simulink model "VehicleDynamics"  (R2025b)
settings: Solver=FixedStepAuto  StartTime=0.0  StopTime=25  FixedStep=0.001  RelTol=1e-3
PreLoadFcn:
  | vehicle_parameters
values from neighbouring files (symbols this model uses):
  beta0 = 0    [vehicle_parameters.m]
  drag = 0    [vehicle_parameters.m]
  ff = 0    [vehicle_parameters.m]
  Fmax = 1274.11    [vehicle_parameters.m]
  N = 15    [MPC_script.m]
  psi0 = 0    [vehicle_parameters.m]
  psi_dot0 = 0    [vehicle_parameters.m]
  RoadCond = 0    [vehicle_parameters.m]
  theta = deg2rad(theta)    [LinearModel.m]    (also in NonLinearModel.m; vehicle_parameters.m = 0)
  vx0 = 0.1    [vehicle_parameters.m]
  vx_constant = 10    [vehicle_parameters.m]
  w = omega_ref    [Fx_w_map.m]
  x0 = 0    [vehicle_parameters.m]
  y0 = 0    [vehicle_parameters.m]
undefined symbols (not defined in the file or in its folder): feedforward, Fx_w_map, K, LinearModel, model, MPC, NonLinearModel, Orientation, Saturation
libraries: slpidlib x1
settings Model: Creator=School  LastModifiedBy=School

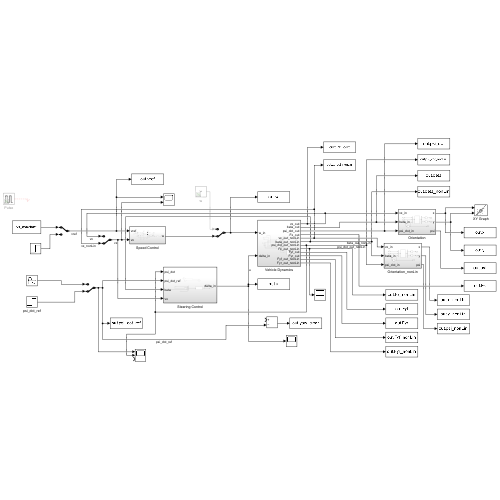
[thumbnail: Simulink's stored preview of the top-level diagram]
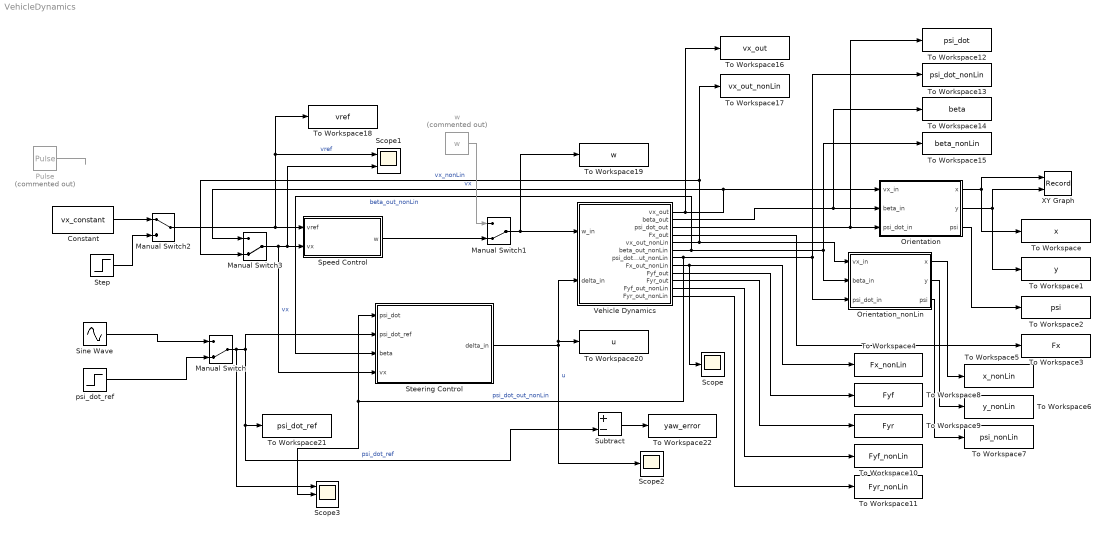
== system VehicleDynamics ==
  Constant : Constant  Value=vx_constant
  Manual Switch : ManualSwitch  CurrentSetting=0
  Manual Switch1 : ManualSwitch  CurrentSetting=0
  Manual Switch2 : ManualSwitch
  Manual Switch3 : ManualSwitch  CurrentSetting=0
  Orientation : Subsystem
  Orientation_nonLin : Subsystem
  Pulse : DiscretePulseGenerator  Commented=on  PulseType=Time based  Amplitude=25  Period=20  PulseWidth=50
  Scope : Scope
      settings: ActiveDisplayYMinimum=-980.76800111578189  ActiveDisplayYMaximum=7754.1424627217448  DataLoggingVariableName=ScopeData5
  Scope1 : Scope  NumInputPorts=2
      settings: ActiveDisplayYMinimum=-1.3886045120699795  ActiveDisplayYMaximum=13.49744060862982  DataLoggingVariableName=ScopeData6
  Scope2 : Scope
      settings: ActiveDisplayYMinimum=-0.012691379481544529  ActiveDisplayYMaximum=0.081489371948126221  DataLoggingVariableName=ScopeData12
  Scope3 : Scope  NumInputPorts=3
      settings: ActiveDisplayYMinimum=-0.011480391205702918  ActiveDisplayYMaximum=0.098238335244763081  DataLoggingVariableName=ScopeData13
  Sine Wave : Sin  Amplitude=deg2rad(5)  Frequency=0.2  SampleTime=0
  Speed Control : Subsystem
  Steering Control : Subsystem
  Step : Step  Time=0  After=10  SampleTime=0
  Subtract : Sum  Inputs=+-
  To Workspace : ToWorkspace  VariableName=x  SaveFormat=Timeseries  SampleTime=-1
  To Workspace1 : ToWorkspace  VariableName=y  SaveFormat=Timeseries  SampleTime=-1
  To Workspace10 : ToWorkspace  VariableName=Fyf_nonLin  SaveFormat=Timeseries  SampleTime=-1
  To Workspace11 : ToWorkspace  VariableName=Fyr_nonLin  SaveFormat=Timeseries  SampleTime=-1
  To Workspace12 : ToWorkspace  VariableName=psi_dot  SaveFormat=Timeseries  SampleTime=-1
  To Workspace13 : ToWorkspace  VariableName=psi_dot_nonLin  SaveFormat=Timeseries  SampleTime=-1
  To Workspace14 : ToWorkspace  VariableName=beta  SaveFormat=Timeseries  SampleTime=-1
  To Workspace15 : ToWorkspace  VariableName=beta_nonLin  SaveFormat=Timeseries  SampleTime=-1
  To Workspace16 : ToWorkspace  VariableName=vx_out  SaveFormat=Timeseries  SampleTime=-1
  To Workspace17 : ToWorkspace  VariableName=vx_out_nonLin  SaveFormat=Timeseries  SampleTime=-1
  To Workspace18 : ToWorkspace  VariableName=vref  SaveFormat=Timeseries  SampleTime=-1
  To Workspace19 : ToWorkspace  VariableName=w  SaveFormat=Timeseries  SampleTime=-1
  To Workspace2 : ToWorkspace  VariableName=psi  SaveFormat=Timeseries  SampleTime=-1
  To Workspace20 : ToWorkspace  VariableName=u  SaveFormat=Timeseries  SampleTime=-1
  To Workspace21 : ToWorkspace  VariableName=psi_dot_ref  SaveFormat=Timeseries  SampleTime=-1
  To Workspace22 : ToWorkspace  VariableName=yaw_error  SaveFormat=Timeseries  SampleTime=-1
  To Workspace3 : ToWorkspace  VariableName=Fx  SaveFormat=Timeseries  SampleTime=-1
  To Workspace4 : ToWorkspace  VariableName=Fx_nonLin  SaveFormat=Timeseries  SampleTime=-1
  To Workspace5 : ToWorkspace  VariableName=x_nonLin  SaveFormat=Timeseries  SampleTime=-1
  To Workspace6 : ToWorkspace  VariableName=y_nonLin  SaveFormat=Timeseries  SampleTime=-1
  To Workspace7 : ToWorkspace  VariableName=psi_nonLin  SaveFormat=Timeseries  SampleTime=-1
  To Workspace8 : ToWorkspace  VariableName=Fyf  SaveFormat=Timeseries  SampleTime=-1
  To Workspace9 : ToWorkspace  VariableName=Fyr  SaveFormat=Timeseries  SampleTime=-1
  Vehicle Dynamics : Subsystem
  XY Graph : Record  NumPorts=2.0  FileSettingsInternal="{\"entries\":[{\"content\":{\"excelSettings\":{\"content\":{},\"type\":\"Streamout.ExcelSettings\"},\"parquetSettings\":{\"content\":{},\"type\":\"Streamout.ParquetSettings\"}},\"type\":\"Streamout.FileSettingStorage\",\"uuid\":\"\"}],\"packageUris\":[\"http:\\/\\/schema.mathworks.com\\/mf0\\/streamout_blocks\\/R2020a\"],\"version\":\"1.0\"}"  FrameSettings=[0, 0]  Layout=[1 1]  SignalsInternal="{\"entries\":[{\"content\":{\"signals\":[{\"content\":{\"blockPath\":[],\"dimensions\":[1,1],\"domain\":\"\",\"lineColor\":\"#ff13a6\",\"lineWidth\":2,\"plots\":[ 1 ],\"port\":1,\"sid\":[\"\"],\"signalID\":1,\"signalName\":\"Orientation:1\"},\"type\":\"RecordBlkView.Signal\",\"uuid\":\"\"},{\"content\":{\"blockPath\":[],\"dimensions\":[1,1],\"domain\":\"\",\"lineColor\":\"#fe330a\",\"lineWidth\":2,\"plots\":[ 1 ],\"port\":2,\"sid\":[\"\"],\"signalID\":2,\"signalName\":\"Orientation:2\"},\"type\":\"RecordBlkView.Signal\",\"uuid\":\"\"}]},\"type\":\"RecordBlkView.InputSignals\",\"uuid\":\"\"}],\"packageUris\":[\"http:\\/\\/schema.mathworks.com\\/mf0\\/streamout_blocks\\/R2020a\"],\"version\":\"1.0\"}"  VisualizationBindings="{\"xyplotplugin\":{\"info\":[{\"series\":[{\"bindingParametersList\":[{\"parameter\":\"X-Axis\",\"signalID\":1,\"signalName\":\"Orientation:1\"},{\"parameter\":\"Y-Axis\",\"signalID\":2,\"signalName\":\"Orientation:2\"}],\"seriesID\":0}],\"subplotID\":1}]}}"  CompatibilityTag=XY
  psi_dot_ref : Step  Time=15  After=deg2rad(5)  SampleTime=0
  w : Constant  Commented=on  Value=w
  wires:
  Vehicle Dynamics/1(vx_out) -> To Workspace16/1, Orientation/1(vx_in), Manual Switch3/1  "vx"
  Vehicle Dynamics/2(beta_out) -> Orientation/2(beta_in), To Workspace14/1
  Vehicle Dynamics/3(psi_dot_out) -> To Workspace12/1, Orientation/3(psi_dot_in)
  Orientation/1(x) -> XY Graph/1, To Workspace/1
  Orientation/2(y) -> XY Graph/2, To Workspace1/1
  Orientation/3(psi) -> To Workspace2/1
  Vehicle Dynamics/4(Fx_out) -> To Workspace3/1
  Vehicle Dynamics/5(vx_out_nonLin) -> Manual Switch3/2, To Workspace17/1, Orientation_nonLin/1(vx_in)  "vx_nonLin"
  Vehicle Dynamics/6(beta_out_nonLin) -> Steering Control/3(beta), To Workspace15/1, Orientation_nonLin/2(beta_in)  "beta_out_nonLin"
  Vehicle Dynamics/7(psi_dot_out_nonLin) -> Scope3/2, Steering Control/1(psi_dot), To Workspace13/1, Orientation_nonLin/3(psi_dot_in)  "psi_dot_out_nonLin"
  Vehicle Dynamics/8(Fx_out_nonLin) -> Scope/1, To Workspace4/1
  Orientation_nonLin/1(x) -> To Workspace5/1
  Orientation_nonLin/2(y) -> To Workspace6/1
  Orientation_nonLin/3(psi) -> To Workspace7/1
  Vehicle Dynamics/9(Fyf_out) -> To Workspace8/1
  Vehicle Dynamics/10(Fyr_out) -> To Workspace9/1
  Vehicle Dynamics/11(Fyf_out_nonLin) -> To Workspace10/1
  Vehicle Dynamics/12(Fyr_out_nonLin) -> To Workspace11/1
  psi_dot_ref/1 -> Manual Switch/2
  w/1 -> Manual Switch1/1
  Manual Switch1/1 -> To Workspace19/1, Vehicle Dynamics/1(w_in)
  Speed Control/1(w) -> Manual Switch1/2
  Pulse/1 -> ?
  Step/1 -> Manual Switch2/2
  Manual Switch3/1 -> Steering Control/4(vx), Scope1/2, Speed Control/2(vx)  "vx"
  Manual Switch2/1 -> Speed Control/1(vref), To Workspace18/1, Scope1/1  "vref"
  Steering Control/1(delta_in) -> Vehicle Dynamics/2(delta_in), To Workspace20/1, Scope2/1  "u"
  Manual Switch/1 -> Scope3/1, Subtract/2, To Workspace21/1, Steering Control/2(psi_dot_ref)  "psi_dot_ref"
  Constant/1 -> Manual Switch2/1
  Subtract/1 -> To Workspace22/1
  Sine Wave/1 -> Manual Switch/1

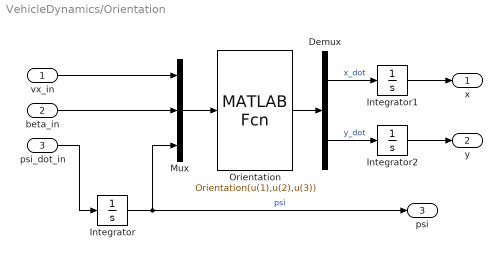
== system VehicleDynamics/Orientation ==
  vx_in : Inport
  beta_in : Inport  Port=2
  psi_dot_in : Inport  Port=3
  Demux : Demux  Outputs=2
  Integrator : Integrator  InitialCondition=psi0
  Integrator1 : Integrator  InitialCondition=x0
  Integrator2 : Integrator  InitialCondition=y0
  Mux : Mux  Inputs=3
  Orientation : MATLABFcn  MATLABFcn=Orientation(u(1),u(2),u(3))  OutputDimensions=[2,1]  Output1D=off
  x : Outport
  y : Outport  Port=2
  psi : Outport  Port=3
  wires:
  Mux/1 -> Orientation/1
  vx_in/1 -> Mux/1
  beta_in/1 -> Mux/2
  Demux/1 -> Integrator1/1  "x_dot"
  Demux/2 -> Integrator2/1  "y_dot"
  Orientation/1 -> Demux/1
  psi_dot_in/1 -> Integrator/1
  Integrator/1 -> Mux/3, psi/1  "psi"
  Integrator2/1 -> y/1
  Integrator1/1 -> x/1

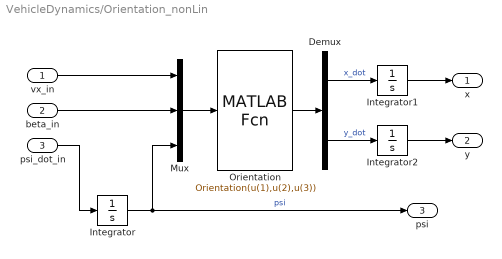
== system VehicleDynamics/Orientation_nonLin ==
  vx_in : Inport
  beta_in : Inport  Port=2
  psi_dot_in : Inport  Port=3
  Demux : Demux  Outputs=2
  Integrator : Integrator  InitialCondition=psi0
  Integrator1 : Integrator  InitialCondition=x0
  Integrator2 : Integrator  InitialCondition=y0
  Mux : Mux  Inputs=3
  Orientation : MATLABFcn  MATLABFcn=Orientation(u(1),u(2),u(3))  OutputDimensions=[2,1]  Output1D=off
  x : Outport
  y : Outport  Port=2
  psi : Outport  Port=3
  wires:
  Mux/1 -> Orientation/1
  vx_in/1 -> Mux/1
  beta_in/1 -> Mux/2
  Demux/1 -> Integrator1/1  "x_dot"
  Demux/2 -> Integrator2/1  "y_dot"
  Orientation/1 -> Demux/1
  psi_dot_in/1 -> Integrator/1
  Integrator/1 -> Mux/3, psi/1  "psi"
  Integrator2/1 -> y/1
  Integrator1/1 -> x/1

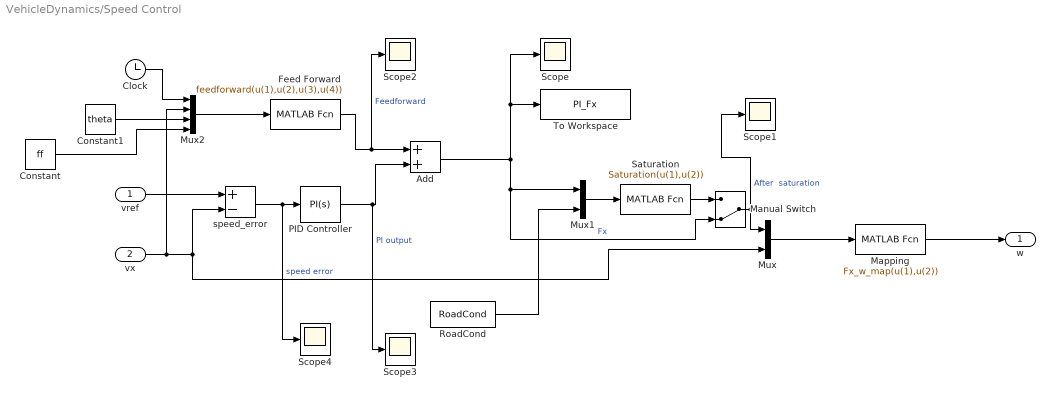
== system VehicleDynamics/Speed Control ==
  vref : Inport
  vx : Inport  Port=2
  Add : Sum
  Clock : Clock
  Constant : Constant  Value=ff
  Constant1 : Constant  Value=theta
  Feed Forward : MATLABFcn  MATLABFcn=feedforward(u(1),u(2),u(3),u(4))  OutputDimensions=1  Output1D=off
  Manual Switch : ManualSwitch  CurrentSetting=0
  Mapping : MATLABFcn  MATLABFcn=Fx_w_map(u(1),u(2))  OutputDimensions=[1,1]  Output1D=off
  Mux : Mux  Inputs=2
  Mux1 : Mux  Inputs=2
  Mux2 : Mux
  PID Controller : slpidlib/PID Controller  Controller=PI  Form=Parallel  TimeDomain=Continuous-time  UseExternalTs=off  SampleTime=-1  IntegratorMethod=Forward Euler  FilterMethod=Forward Euler  ControllerParametersSource=internal  P=4*206  I=206  UseKiTs=off  D=0  UseExternalDerivativeSource=off  N=100  UseFilter=on  TunerSelectOption=Transfer Function Based (PID Tuner App)  InitialConditionSource=internal  InitialConditionForIntegrator=0  InitialConditionForFilter=0  DifferentiatorICPrevScaledInput=0  ExternalReset=none  TrackingMode=off  Kt=1  LimitOutput=on  SatLimitsSource=internal  UpperSaturationLimit=Fmax  LowerSaturationLimit=-Fmax  LinearizeAsGain=off  AntiWindupMode=back-calculation  Kb=206/(4*206)  LimitIntegrator=off  UpperIntegratorSaturationLimit=inf  LowerIntegratorSaturationLimit=-inf  POutMin=[]  POutMax=[]  IOutMin=[]  IOutMax=[]  DOutMin=[]  DOutMax=[]  NOutMin=[]  NOutMax=[]  SumOutMin=[]  SumOutMax=[]  SaturationOutMin=[]  SaturationOutMax=[]  PParamMin=[]  PParamMax=[]  IParamMin=[]  IParamMax=[]  DParamMin=[]  DParamMax=[]  NParamMin=[]  NParamMax=[]  KbParamMin=[]  KbParamMax=[]  KtParamMin=[]  KtParamMax=[]  KbOutMin=[]  KbOutMax=[]  KtOutMin=[]  KtOutMax=[]  IntegratorOutMin=[]  IntegratorOutMax=[]  FilterOutMin=[]  FilterOutMax=[]  SumI1OutMin=[]  SumI1OutMax=[]  SumI2OutMin=[]  SumI2OutMax=[]  SumI3OutMin=[]  SumI3OutMax=[]  SumI4OutMin=[]  SumI4OutMax=[]  SumDOutMin=[]  SumDOutMax=[]  DifferentiatorOutMin=[]  DifferentiatorOutMax=[]  FilterDiffOutCoefMin=[]  FilterDiffOutCoefMax=[]  ReciprocalOutMin=[]  ReciprocalOutMax=[]  SumDenOutMin=[]  SumDenOutMax=[]  SumNumOutMin=[]  SumNumOutMax=[]  DivideOutMin=[]  DivideOutMax=[]  UdiffTsProdOutMin=[]  UdiffTsProdOutMax=[]  NTsProdOutMin=[]  NTsProdOutMax=[]  UintegralTsProdOutMin=[]  UintegralTsProdOutMax=[]  UngainTsProdOutMin=[]  UngainTsProdOutMax=[]  ClampingZeroOutDataTypeStr=Inherit: Inherit via back propagation  ClampingZeroOutMin=[]  ClampingZeroOutMax=[]  FilterDenConstantOutDataTypeStr=Inherit: Inherit via back propagation  FilterDenConstantOutMin=[]  FilterDenConstantOutMax=[]  PCopyOutDataTypeStr=Inherit: Inherit via back propagation  PCopyOutMin=[]  PCopyOutMax=[]  NCopyOutDataTypeStr=Inherit: Inherit via back propagation  NCopyOutMin=[]  NCopyOutMax=[]  IntegratorContinuousStateAttributes=''  IntegratorStateMustResolveToSignalObject=off  IntegratorRTWStateStorageClass=Auto  FilterContinuousStateAttributes=''  FilterStateMustResolveToSignalObject=off  FilterRTWStateStorageClass=Auto  ParallelPVariant=InternalParameters  IdealPVariant=Disabled  IVariant=InternalParameters  DVariant=Disabled  IntegratorVariant=Continuous  SatVariant=Enabled  AWVariant=BackCalculation  PCopyVariant=Disabled  TRVariant=Disabled  FdbkBlocksVariant=Forward  IdealPFdbkVariant=Disabled  SatFdbkVariant=Disabled  DerivativeFilterVariant=Disabled  NVariant=Disabled  NCopyVariant=Disabled_SignalSpec  FilterICVariant=Disabled  IntegratorICVariant=InternalICs  ExternalResetVariant=Disabled  TRSumVariant=Passthrough  SumFdbkVariant=Disabled  SumVariant=Sum_PI  TsampFilterVariant=InternalTs  TsampNgainVariant=Passthrough  TsampIntegralVariant=Disabled_SignalSpec  ExternalSaturationOutDataTypeStr=Inherit: Same as second input  DerivativeSourceVariant=Disabled  PreIntVariant=InternalPreInt
  RoadCond : Constant  Value=RoadCond
  Saturation : MATLABFcn  MATLABFcn=Saturation(u(1),u(2))  OutputDimensions=1  Output1D=off
  Scope{,1..4} (5 alike) : Scope
      Scope settings: ActiveDisplayYMinimum=-1555.3315998720143  ActiveDisplayYMaximum=12511.361836654254  DataLoggingVariableName=ScopeData7
      Scope1 settings: ActiveDisplayYMinimum=-1027.3262882468107  ActiveDisplayYMaximum=7759.3140320274233  DataLoggingVariableName=ScopeData8
      Scope2 settings: ActiveDisplayYMinimum=1496.5482656031122  ActiveDisplayYMaximum=2205.6055136294681  DataLoggingVariableName=ScopeData9
      Scope3 settings: ActiveDisplayYMinimum=-2981.7756192687925  ActiveDisplayYMaximum=7976.4750688076438  DataLoggingVariableName=ScopeData10
      Scope4 settings: ActiveDisplayYMinimum=-10.514371710749185  ActiveDisplayYMaximum=34.390485745638792  DataLoggingVariableName=ScopeData11
  To Workspace : ToWorkspace  VariableName=PI_Fx  SaveFormat=Timeseries  SampleTime=-1
  speed_error : Sum  Inputs=+-
  w : Outport
  wires:
  vref/1 -> speed_error/1
  vx/1 -> Mux2/2, Mux/2, speed_error/2
  speed_error/1 -> PID Controller/1, Scope4/1  "speed error"
  Mux/1 -> Mapping/1
  Mapping/1 -> w/1
  Mux1/1 -> Saturation/1
  RoadCond/1 -> Mux1/2
  Saturation/1 -> Manual Switch/1
  Manual Switch/1 -> Mux/1, Scope1/1  "After  saturation"
  PID Controller/1 -> Scope3/1, Add/2  "PI output"
  Add/1 -> Scope/1, To Workspace/1, Manual Switch/2, Mux1/1  "Fx"
  Feed Forward/1 -> Scope2/1, Add/1  "Feedforward"
  Constant/1 -> Mux2/4
  Mux2/1 -> Feed Forward/1
  Clock/1 -> Mux2/1
  Constant1/1 -> Mux2/3

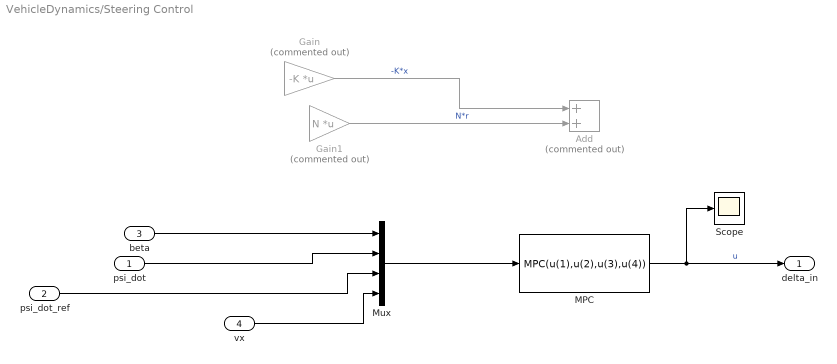
== system VehicleDynamics/Steering Control ==
  psi_dot : Inport
  psi_dot_ref : Inport  Port=2
  beta : Inport  Port=3
  vx : Inport  Port=4
  Add : Sum  Commented=on
  Gain : Gain  Commented=on  Gain=-K  Multiplication=Matrix(K*u)
  Gain1 : Gain  Commented=on  Gain=N  Multiplication=Matrix(K*u)
  MPC : MATLABFcn  MATLABFcn=MPC(u(1),u(2),u(3),u(4))  OutputDimensions=1  Output1D=off
  Mux : Mux
  Scope : Scope
      settings: ActiveDisplayYMinimum=-1  ActiveDisplayYMaximum=1  DataLoggingVariableName=ScopeData14
  delta_in : Outport
  wires:
  psi_dot/1 -> Mux/2
  beta/1 -> Mux/1
  Gain/1 -> Add/1  "-K*x"
  Gain1/1 -> Add/2  "N*r"
  MPC/1 -> Scope/1, delta_in/1  "u"
  psi_dot_ref/1 -> Mux/3
  vx/1 -> Mux/4
  Mux/1 -> MPC/1

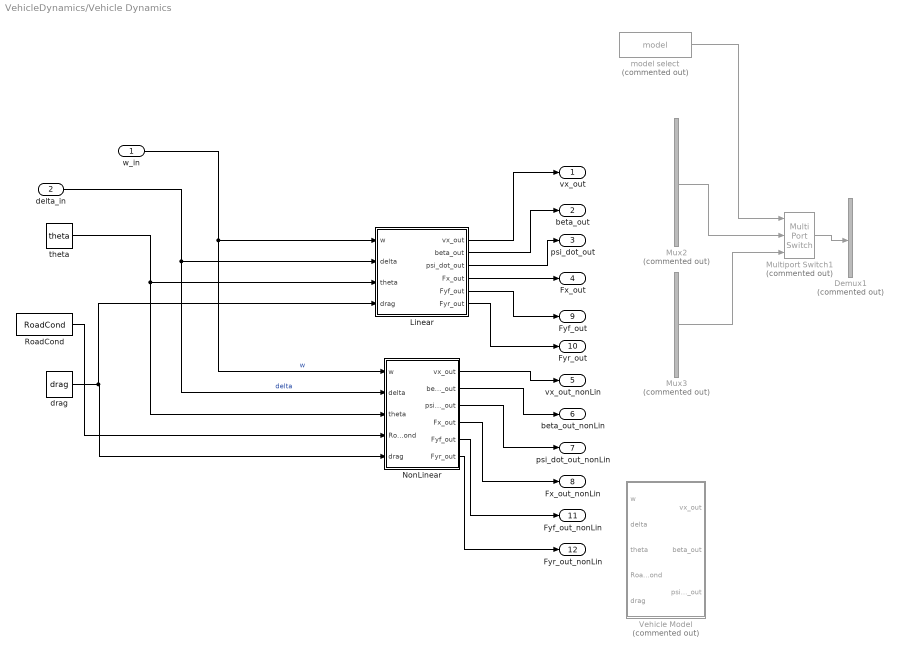
== system VehicleDynamics/Vehicle Dynamics ==
  w_in : Inport
  delta_in : Inport  Port=2
  Demux1 : Demux  Commented=on
  Linear : Subsystem
  Multiport Switch1 : MultiPortSwitch  Commented=on  Inputs=2  SaturateOnIntegerOverflow=off  InputSameDT=off
  Mux2 : Mux  Commented=on
  Mux3 : Mux  Commented=on
  NonLinear : Subsystem
  RoadCond : Constant  Value=RoadCond
  Vehicle Model : Subsystem  Commented=on  Variant=on
  drag : Constant  Value=drag
  model select : Constant  Commented=on  Value=model
  theta : Constant  Value=theta
  vx_out : Outport
  beta_out : Outport  Port=2
  psi_dot_out : Outport  Port=3
  Fx_out : Outport  Port=4
  vx_out_nonLin : Outport  Port=5
  beta_out_nonLin : Outport  Port=6
  psi_dot_out_nonLin : Outport  Port=7
  Fx_out_nonLin : Outport  Port=8
  Fyf_out : Outport  Port=9
  Fyr_out : Outport  Port=10
  Fyf_out_nonLin : Outport  Port=11
  Fyr_out_nonLin : Outport  Port=12
  wires:
  w_in/1 -> NonLinear/1(w), Linear/1(w)  "w"
  delta_in/1 -> NonLinear/2(delta), Linear/2(delta)  "delta"
  theta/1 -> NonLinear/3(theta), Linear/3(theta)
  RoadCond/1 -> NonLinear/4(RoadCond)
  drag/1 -> Linear/4(drag), NonLinear/5(drag)
  Multiport Switch1/1 -> Demux1/1
  model select/1 -> Multiport Switch1/1
  Mux2/1 -> Multiport Switch1/2
  Mux3/1 -> Multiport Switch1/3
  Linear/1(vx_out) -> vx_out/1
  Linear/2(beta_out) -> beta_out/1
  Linear/3(psi_dot_out) -> psi_dot_out/1
  Linear/4(Fx_out) -> Fx_out/1
  NonLinear/1(vx_out) -> vx_out_nonLin/1
  NonLinear/2(beta_out) -> beta_out_nonLin/1
  NonLinear/3(psi_dot_out) -> psi_dot_out_nonLin/1
  NonLinear/4(Fx_out) -> Fx_out_nonLin/1
  Linear/5(Fyf_out) -> Fyf_out/1
  Linear/6(Fyr_out) -> Fyr_out/1
  NonLinear/5(Fyf_out) -> Fyf_out_nonLin/1
  NonLinear/6(Fyr_out) -> Fyr_out_nonLin/1

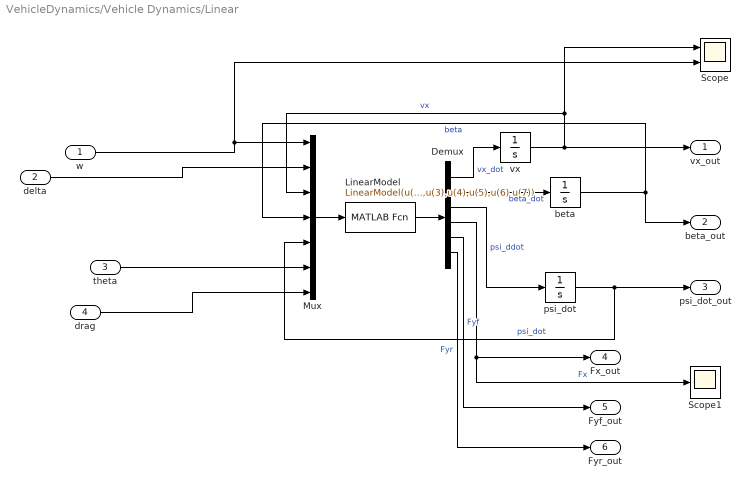
== system VehicleDynamics/Vehicle Dynamics/Linear ==
  w : Inport
  delta : Inport  Port=2
  theta : Inport  Port=3
  drag : Inport  Port=4
  Demux : Demux  Outputs=6
  LinearModel : MATLABFcn  MATLABFcn=LinearModel(u(1),u(2),u(3),u(4),u(5),u(6),u(7))  OutputDimensions=[6,1]  Output1D=off
  Mux : Mux  Inputs=7
  Scope : Scope  NumInputPorts=2
      settings: ActiveDisplayYMinimum=-3.6374999999999993  ActiveDisplayYMaximum=33.7375  DataLoggingVariableName=ScopeData2
  Scope1 : Scope
      settings: ActiveDisplayYMinimum=-735634.97602375317  ActiveDisplayYMaximum=6.61829277511375E+6  DataLoggingVariableName=ScopeData3
  beta : Integrator  InitialCondition=beta0
  psi_dot : Integrator  InitialCondition=psi_dot0
  vx : Integrator  InitialCondition=vx0
  vx_out : Outport
  beta_out : Outport  Port=2
  psi_dot_out : Outport  Port=3
  Fx_out : Outport  Port=4
  Fyf_out : Outport  Port=5
  Fyr_out : Outport  Port=6
  wires:
  delta/1 -> Mux/2
  w/1 -> Scope/2, Mux/1
  psi_dot/1 -> psi_dot_out/1, Mux/5  "psi_dot"
  LinearModel/1 -> Demux/1
  vx/1 -> vx_out/1, Scope/1, Mux/3  "vx"
  Demux/1 -> vx/1  "vx_dot"
  Demux/2 -> beta/1  "beta_dot"
  theta/1 -> Mux/6
  drag/1 -> Mux/7
  Mux/1 -> LinearModel/1
  Demux/3 -> psi_dot/1  "psi_ddot"
  beta/1 -> beta_out/1, Mux/4  "beta"
  Demux/4 -> Scope1/1, Fx_out/1  "Fx"
  Demux/5 -> Fyf_out/1  "Fyf"
  Demux/6 -> Fyr_out/1  "Fyr"

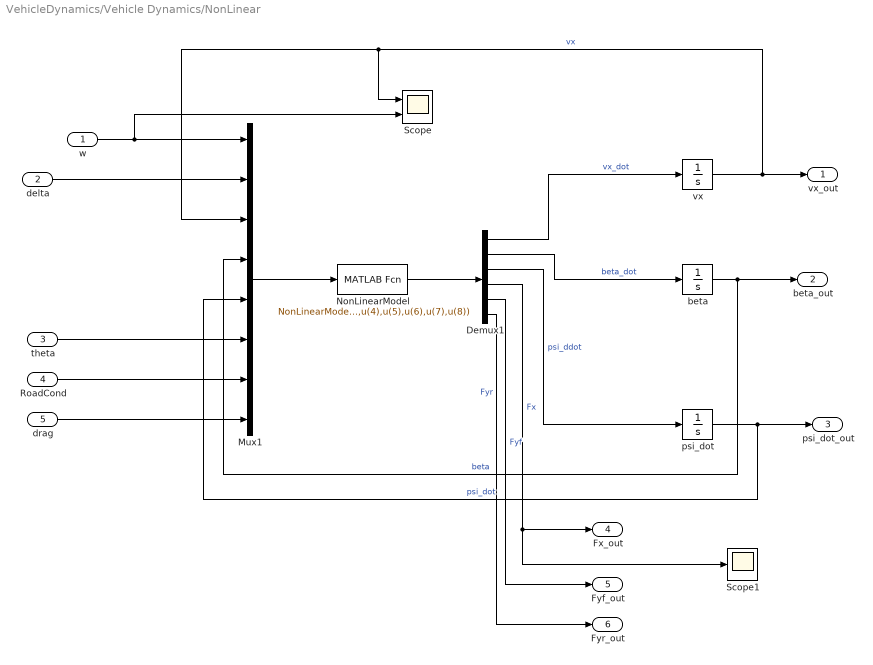
== system VehicleDynamics/Vehicle Dynamics/NonLinear ==
  w : Inport
  delta : Inport  Port=2
  theta : Inport  Port=3
  RoadCond : Inport  Port=4
  drag : Inport  Port=5
  Demux1 : Demux  Outputs=6
  Mux1 : Mux  Inputs=8
  NonLinearModel : MATLABFcn  MATLABFcn=NonLinearModel(u(1),u(2),u(3),u(4),u(5),u(6),u(7),u(8))  OutputDimensions=[6,1]  Output1D=off
  Scope : Scope  NumInputPorts=2
      settings: ActiveDisplayYMinimum=-3.6374999999999993  ActiveDisplayYMaximum=33.7375
  Scope1 : Scope
      settings: ActiveDisplayYMinimum=-2.1063877440902755E+7  ActiveDisplayYMaximum=8.0749890326656476E+6  DataLoggingVariableName=ScopeData4
  beta : Integrator  InitialCondition=beta0
  psi_dot : Integrator  InitialCondition=psi_dot0
  vx : Integrator  InitialCondition=vx0
  vx_out : Outport
  beta_out : Outport  Port=2
  psi_dot_out : Outport  Port=3
  Fx_out : Outport  Port=4
  Fyf_out : Outport  Port=5
  Fyr_out : Outport  Port=6
  wires:
  drag/1 -> Mux1/8
  Mux1/1 -> NonLinearModel/1
  RoadCond/1 -> Mux1/7
  NonLinearModel/1 -> Demux1/1
  delta/1 -> Mux1/2
  Demux1/3 -> psi_dot/1  "psi_ddot"
  theta/1 -> Mux1/6
  Demux1/2 -> beta/1  "beta_dot"
  Demux1/1 -> vx/1  "vx_dot"
  beta/1 -> beta_out/1, Mux1/4  "beta"
  vx/1 -> vx_out/1, Scope/1, Mux1/3  "vx"
  w/1 -> Scope/2, Mux1/1
  psi_dot/1 -> psi_dot_out/1, Mux1/5  "psi_dot"
  Demux1/4 -> Fx_out/1, Scope1/1  "Fx"
  Demux1/5 -> Fyf_out/1  "Fyf"
  Demux1/6 -> Fyr_out/1  "Fyr"

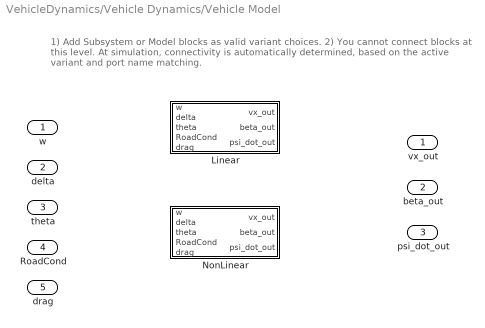
== system VehicleDynamics/Vehicle Dynamics/Vehicle Model ==
  note: 1) Add Subsystem or Model blocks as valid variant choices.
      | 2) You cannot connect blocks at this level. At simulation, connectivity is automatically
      | determined, based on the active variant and port name matching.
  w : Inport
  delta : Inport  Port=2
  theta : Inport  Port=3
  RoadCond : Inport  Port=4
  drag : Inport  Port=5
  Linear : Subsystem  VariantControl=true
  NonLinear : Subsystem  VariantControl=false
  vx_out : Outport
  beta_out : Outport  Port=2
  psi_dot_out : Outport  Port=3

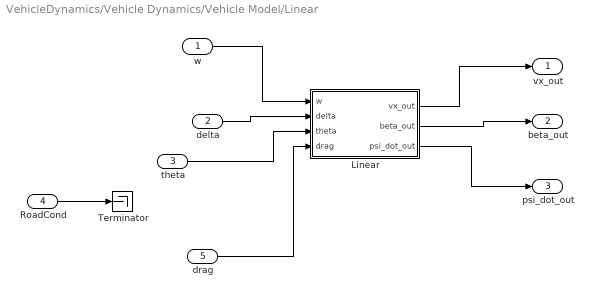
== system VehicleDynamics/Vehicle Dynamics/Vehicle Model/Linear ==
  w : Inport
  delta : Inport  Port=2
  theta : Inport  Port=3
  RoadCond : Inport  Port=4
  drag : Inport  Port=5
  Linear : Subsystem
  Terminator : Terminator
  vx_out : Outport
  beta_out : Outport  Port=2
  psi_dot_out : Outport  Port=3
  wires:
  w/1 -> Linear/1(w)
  delta/1 -> Linear/2(delta)
  theta/1 -> Linear/3(theta)
  Linear/1(vx_out) -> vx_out/1
  Linear/2(beta_out) -> beta_out/1
  Linear/3(psi_dot_out) -> psi_dot_out/1
  drag/1 -> Linear/4(drag)
  RoadCond/1 -> Terminator/1

== system VehicleDynamics/Vehicle Dynamics/Vehicle Model/NonLinear ==
  w : Inport
  delta : Inport  Port=2
  theta : Inport  Port=3
  RoadCond : Inport  Port=4
  drag : Inport  Port=5
  NonLinear : Subsystem
  vx_out : Outport
  beta_out : Outport  Port=2
  psi_dot_out : Outport  Port=3
  wires:
  w/1 -> NonLinear/1(w)
  delta/1 -> NonLinear/2(delta)
  theta/1 -> NonLinear/3(theta)
  RoadCond/1 -> NonLinear/4(RoadCond)
  drag/1 -> NonLinear/5(drag)
  NonLinear/2(beta_out) -> beta_out/1
  NonLinear/1(vx_out) -> vx_out/1
  NonLinear/3(psi_dot_out) -> psi_dot_out/1

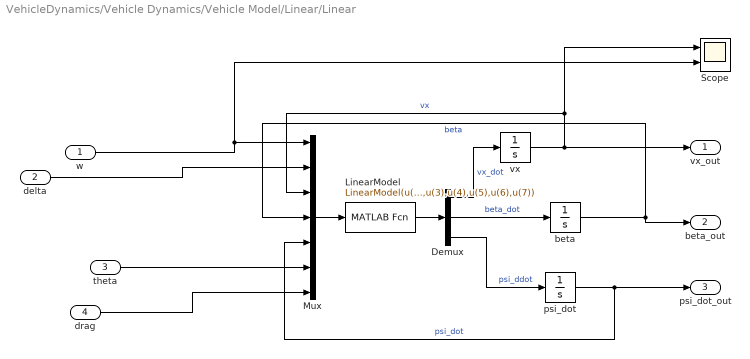
== system VehicleDynamics/Vehicle Dynamics/Vehicle Model/Linear/Linear ==
  w : Inport
  delta : Inport  Port=2
  theta : Inport  Port=3
  drag : Inport  Port=4
  Demux : Demux  Outputs=3
  LinearModel : MATLABFcn  MATLABFcn=LinearModel(u(1),u(2),u(3),u(4),u(5),u(6),u(7))  OutputDimensions=[3,1]  Output1D=off
  Mux : Mux  Inputs=7
  Scope : Scope  NumInputPorts=2
      settings: ActiveDisplayYMinimum=-3.6374999999999993  ActiveDisplayYMaximum=33.7375
  beta : Integrator  InitialCondition=beta0
  psi_dot : Integrator  InitialCondition=psi_dot0
  vx : Integrator  InitialCondition=vx0
  vx_out : Outport
  beta_out : Outport  Port=2
  psi_dot_out : Outport  Port=3
  wires:
  psi_dot/1 -> psi_dot_out/1, Mux/5  "psi_dot"
  theta/1 -> Mux/6
  beta/1 -> beta_out/1, Mux/4  "beta"
  vx/1 -> vx_out/1, Scope/1, Mux/3  "vx"
  Demux/3 -> psi_dot/1  "psi_ddot"
  Mux/1 -> LinearModel/1
  Demux/1 -> vx/1  "vx_dot"
  w/1 -> Scope/2, Mux/1
  LinearModel/1 -> Demux/1
  Demux/2 -> beta/1  "beta_dot"
  delta/1 -> Mux/2
  drag/1 -> Mux/7

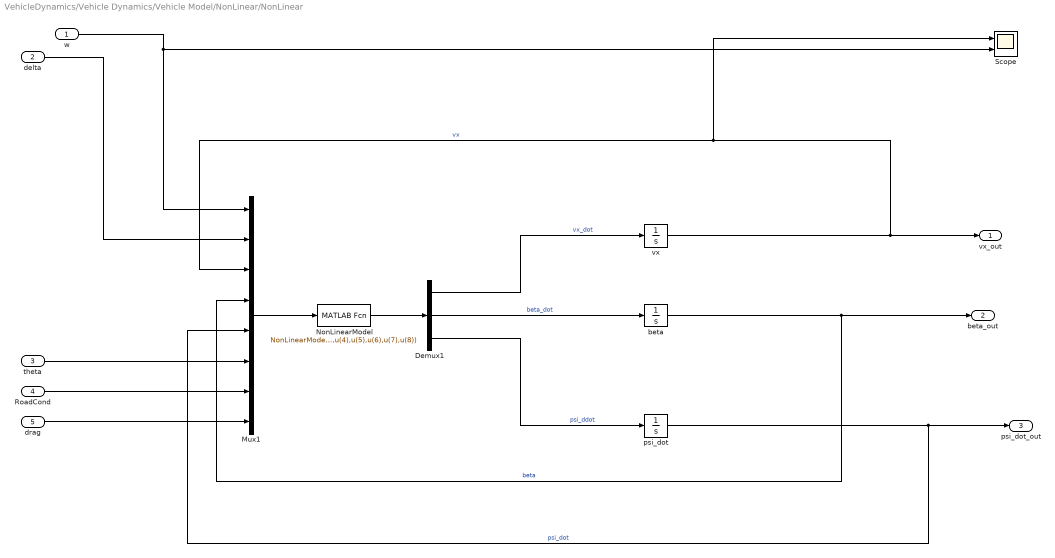
== system VehicleDynamics/Vehicle Dynamics/Vehicle Model/NonLinear/NonLinear ==
  w : Inport
  delta : Inport  Port=2
  theta : Inport  Port=3
  RoadCond : Inport  Port=4
  drag : Inport  Port=5
  Demux1 : Demux  Outputs=3
  Mux1 : Mux  Inputs=8
  NonLinearModel : MATLABFcn  MATLABFcn=NonLinearModel(u(1),u(2),u(3),u(4),u(5),u(6),u(7),u(8))  OutputDimensions=[3,1]  Output1D=off
  Scope : Scope  NumInputPorts=2
      settings: ActiveDisplayYMinimum=-3.6374999999999993  ActiveDisplayYMaximum=33.7375
  beta : Integrator  InitialCondition=beta0
  psi_dot : Integrator  InitialCondition=psi_dot0
  vx : Integrator  InitialCondition=vx0
  vx_out : Outport
  beta_out : Outport  Port=2
  psi_dot_out : Outport  Port=3
  wires:
  drag/1 -> Mux1/8
  Mux1/1 -> NonLinearModel/1
  RoadCond/1 -> Mux1/7
  NonLinearModel/1 -> Demux1/1
  delta/1 -> Mux1/2
  Demux1/3 -> psi_dot/1  "psi_ddot"
  theta/1 -> Mux1/6
  Demux1/2 -> beta/1  "beta_dot"
  Demux1/1 -> vx/1  "vx_dot"
  beta/1 -> beta_out/1, Mux1/4  "beta"
  vx/1 -> Scope/1, Mux1/3, vx_out/1  "vx"
  w/1 -> Mux1/1, Scope/2
  psi_dot/1 -> psi_dot_out/1, Mux1/5  "psi_dot"
